simulink model "arducopter"  (R2024b)
settings: Solver=FixedStepAuto  StartTime=0.0  StopTime=simIn.param.timeEnd  FixedStep=simIn.param.dt  RelTol=1e-3
undefined symbols (not defined in the file or in its folder): DiscIntNeverNeededParam, sim, simIn
libraries: simulink x60, slident x4, vrlib x1
(part 2 of 9)

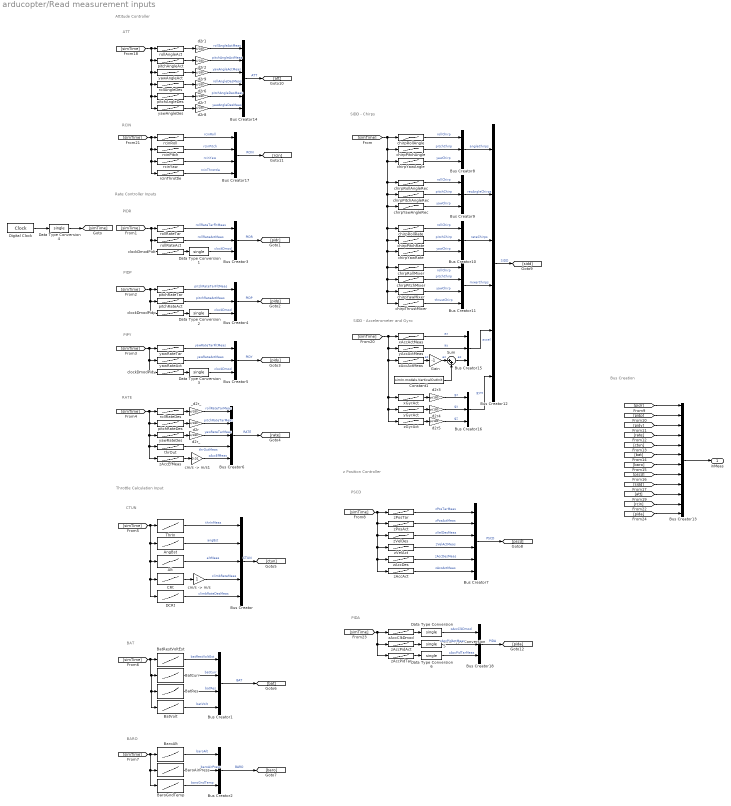
== system arducopter/Read measurement inputs ==
  note: PIDA
  note: Rate Controller Inputs
  note: SIDD - Chirps
  note: PIDR
  note: PIDP
  note: PIPY
  note: RATE
  note: CTUN
  note: BAT
  note: BARO
  note: Throttle Calculation Input
  note: PSCD
  note: z Position Controller
  note: Bus Creation
  note: ATT
  note: Attitude Controller
  note: SIDD - Accelerometer and Gyro
  note: RCIN
  Alt : Lookup_n-D  NumberOfTableDimensions=1  BreakpointsForDimension1=simIn.signals.CTUN.Time  Table=simIn.signals.CTUN.Alt  TableDataTypeStr=single  InternalRulePriority=Speed  OutDataTypeStr=Inherit: Inherit from 'Table data'  RndMeth=Simplest
  AngBst : Lookup_n-D  NumberOfTableDimensions=1  BreakpointsForDimension1=simIn.signals.CTUN.Time  Table=simIn.signals.CTUN.AngBst  TableDataTypeStr=single  InternalRulePriority=Speed  OutDataTypeStr=Inherit: Inherit from 'Table data'  RndMeth=Simplest
  BaroAirPress : Lookup_n-D  NumberOfTableDimensions=1  BreakpointsForDimension1=simIn.signals.BARO.Time  Table=simIn.signals.BARO.AirPress  TableDataTypeStr=Inherit: Inherit from 'Table data'  InternalRulePriority=Speed  OutDataTypeStr=Inherit: Inherit from 'Table data'  RndMeth=Simplest
  BaroAlt : Lookup_n-D  NumberOfTableDimensions=1  BreakpointsForDimension1=simIn.signals.BARO.Time  Table=simIn.signals.BARO.Alt  TableDataTypeStr=Inherit: Inherit from 'Table data'  InternalRulePriority=Speed  OutDataTypeStr=Inherit: Inherit from 'Table data'  RndMeth=Simplest
  BaroGndTemp : Lookup_n-D  NumberOfTableDimensions=1  BreakpointsForDimension1=simIn.signals.BARO.Time  Table=simIn.signals.BARO.GndTemp  TableDataTypeStr=Inherit: Inherit from 'Table data'  InternalRulePriority=Speed  OutDataTypeStr=Inherit: Inherit from 'Table data'  RndMeth=Simplest
  BatCurr : Lookup_n-D  NumberOfTableDimensions=1  BreakpointsForDimension1=simIn.signals.BAT.Time  Table=simIn.signals.BAT.Curr  TableDataTypeStr=single  InternalRulePriority=Speed  OutDataTypeStr=Inherit: Inherit from 'Table data'  RndMeth=Simplest
  BatRes : Lookup_n-D  NumberOfTableDimensions=1  BreakpointsForDimension1=simIn.signals.BAT.Time  Table=simIn.signals.BAT.Res  TableDataTypeStr=single  InternalRulePriority=Speed  OutDataTypeStr=Inherit: Inherit from 'Table data'  RndMeth=Simplest
  BatRestVoltEst : Lookup_n-D  NumberOfTableDimensions=1  BreakpointsForDimension1=simIn.signals.BAT.Time  Table=simIn.signals.BAT.RestVoltEst  TableDataTypeStr=single  InternalRulePriority=Speed  OutDataTypeStr=Inherit: Inherit from 'Table data'  RndMeth=Simplest
  BatVolt : Lookup_n-D  NumberOfTableDimensions=1  BreakpointsForDimension1=simIn.signals.BAT.Time  Table=simIn.signals.BAT.Volt  TableDataTypeStr=Inherit: Inherit from 'Table data'  InternalRulePriority=Speed  OutDataTypeStr=Inherit: Inherit from 'Table data'  RndMeth=Simplest
  Bus Creator : BusCreator  Inputs=5
  Bus Creator1 : BusCreator  Inputs=4
  Bus Creator{2..5,8..10,15..16,18} (10 alike) : BusCreator  Inputs=3
  Bus Creator11 : BusCreator  Inputs=4
  Bus Creator12 : BusCreator  Inputs=6
  Bus Creator13 : BusCreator  Inputs=12
  Bus Creator14 : BusCreator  Inputs=6
  Bus Creator17 : BusCreator  Inputs=4
  Bus Creator6 : BusCreator  Inputs=5
  Bus Creator7 : BusCreator  Inputs=6
  CRt : Lookup_n-D  NumberOfTableDimensions=1  BreakpointsForDimension1=simIn.signals.CTUN.Time  Table=simIn.signals.CTUN.CRt  TableDataTypeStr=single  InternalRulePriority=Speed  OutDataTypeStr=Inherit: Inherit from 'Table data'  RndMeth=Simplest
  Constant1 : Constant  Value=simIn.models.VerticalOutInit
  DCRt : Lookup_n-D  NumberOfTableDimensions=1  BreakpointsForDimension1=simIn.signals.CTUN.Time  Table=simIn.signals.CTUN.DCRt  TableDataTypeStr=single  InternalRulePriority=Speed  OutDataTypeStr=Inherit: Inherit from 'Table data'  RndMeth=Simplest
  Data Type Conversion{,1..6} (7 alike) : DataTypeConversion  OutDataTypeStr=single  SaturateOnIntegerOverflow=off  RndMeth=Floor
  Digital Clock : DigitalClock  SampleTime=simIn.param.dt
  Gain : Gain  Gain=-1
  Sum : Sum  Inputs=|++
  ThrIn : Lookup_n-D  NumberOfTableDimensions=1  BreakpointsForDimension1=simIn.signals.CTUN.Time  Table=simIn.signals.CTUN.ThrIn  TableDataTypeStr=single  InternalRulePriority=Speed  OutDataTypeStr=Inherit: Inherit from 'Table data'  RndMeth=Simplest
  _d2r_ : Gain  Gain=pi/180
  chirpPitchAngle : Lookup_n-D  NumberOfTableDimensions=1  BreakpointsForDimension1=simIn.signals.SIDD.Time{2}  Table=simIn.signals.SIDD.Chirp{2}  TableDataTypeStr=Inherit: Inherit from 'Table data'  InternalRulePriority=Speed  OutDataTypeStr=Inherit: Inherit from 'Table data'  RndMeth=Simplest
  chirpPitchAngleRec : Lookup_n-D  NumberOfTableDimensions=1  BreakpointsForDimension1=simIn.signals.SIDD.Time{5}  Table=simIn.signals.SIDD.Chirp{5}  TableDataTypeStr=Inherit: Inherit from 'Table data'  InternalRulePriority=Speed  OutDataTypeStr=Inherit: Inherit from 'Table data'  RndMeth=Simplest
  chirpPitchMixer : Lookup_n-D  NumberOfTableDimensions=1  BreakpointsForDimension1=simIn.signals.SIDD.Time{11}  Table=simIn.signals.SIDD.Chirp{11}  TableDataTypeStr=Inherit: Inherit from 'Table data'  InternalRulePriority=Speed  OutDataTypeStr=Inherit: Inherit from 'Table data'  RndMeth=Simplest
  chirpPitchRate : Lookup_n-D  NumberOfTableDimensions=1  BreakpointsForDimension1=simIn.signals.SIDD.Time{8}  Table=simIn.signals.SIDD.Chirp{8}  TableDataTypeStr=Inherit: Inherit from 'Table data'  InternalRulePriority=Speed  OutDataTypeStr=Inherit: Inherit from 'Table data'  RndMeth=Simplest
  chirpRollAngle : Lookup_n-D  NumberOfTableDimensions=1  BreakpointsForDimension1=simIn.signals.SIDD.Time{1}  Table=simIn.signals.SIDD.Chirp{1}  TableDataTypeStr=Inherit: Inherit from 'Table data'  InternalRulePriority=Speed  OutDataTypeStr=Inherit: Inherit from 'Table data'  RndMeth=Simplest
  chirpRollAngleRec : Lookup_n-D  NumberOfTableDimensions=1  BreakpointsForDimension1=simIn.signals.SIDD.Time{4}  Table=simIn.signals.SIDD.Chirp{4}  TableDataTypeStr=Inherit: Inherit from 'Table data'  InternalRulePriority=Speed  OutDataTypeStr=Inherit: Inherit from 'Table data'  RndMeth=Simplest
  chirpRollMixer : Lookup_n-D  NumberOfTableDimensions=1  BreakpointsForDimension1=simIn.signals.SIDD.Time{10}  Table=simIn.signals.SIDD.Chirp{10}  TableDataTypeStr=Inherit: Inherit from 'Table data'  InternalRulePriority=Speed  OutDataTypeStr=Inherit: Inherit from 'Table data'  RndMeth=Simplest
  chirpRollRate : Lookup_n-D  NumberOfTableDimensions=1  BreakpointsForDimension1=simIn.signals.SIDD.Time{7}  Table=simIn.signals.SIDD.Chirp{7}  TableDataTypeStr=Inherit: Inherit from 'Table data'  InternalRulePriority=Speed  OutDataTypeStr=Inherit: Inherit from 'Table data'  RndMeth=Simplest
  chirpThrustMixer : Lookup_n-D  NumberOfTableDimensions=1  BreakpointsForDimension1=simIn.signals.SIDD.Time{13}  Table=simIn.signals.SIDD.Chirp{13}  TableDataTypeStr=Inherit: Inherit from 'Table data'  InternalRulePriority=Speed  OutDataTypeStr=Inherit: Inherit from 'Table data'  RndMeth=Simplest
  chirpYawAngle : Lookup_n-D  NumberOfTableDimensions=1  BreakpointsForDimension1=simIn.signals.SIDD.Time{3}  Table=simIn.signals.SIDD.Chirp{3}  TableDataTypeStr=Inherit: Inherit from 'Table data'  InternalRulePriority=Speed  OutDataTypeStr=Inherit: Inherit from 'Table data'  RndMeth=Simplest
  chirpYawAngleRec : Lookup_n-D  NumberOfTableDimensions=1  BreakpointsForDimension1=simIn.signals.SIDD.Time{6}  Table=simIn.signals.SIDD.Chirp{6}  TableDataTypeStr=Inherit: Inherit from 'Table data'  InternalRulePriority=Speed  OutDataTypeStr=Inherit: Inherit from 'Table data'  RndMeth=Simplest
  chirpYawMixer : Lookup_n-D  NumberOfTableDimensions=1  BreakpointsForDimension1=simIn.signals.SIDD.Time{12}  Table=simIn.signals.SIDD.Chirp{12}  TableDataTypeStr=Inherit: Inherit from 'Table data'  InternalRulePriority=Speed  OutDataTypeStr=Inherit: Inherit from 'Table data'  RndMeth=Simplest
  chirpYawRate : Lookup_n-D  NumberOfTableDimensions=1  BreakpointsForDimension1=simIn.signals.SIDD.Time{9}  Table=simIn.signals.SIDD.Chirp{9}  TableDataTypeStr=Inherit: Inherit from 'Table data'  InternalRulePriority=Speed  OutDataTypeStr=Inherit: Inherit from 'Table data'  RndMeth=Simplest
  clockDmodPidp : Lookup_n-D  NumberOfTableDimensions=1  BreakpointsForDimension1=simIn.signals.PIDP.Time  Table=simIn.signals.PIDP.ClockDMod  InternalRulePriority=Speed  RndMeth=Simplest
  clockDmodPidr : Lookup_n-D  NumberOfTableDimensions=1  BreakpointsForDimension1=simIn.signals.PIDR.Time  Table=simIn.signals.PIDR.ClockDMod  TableDataTypeStr=Inherit: Inherit from 'Table data'  InternalRulePriority=Speed  OutDataTypeStr=Inherit: Inherit from 'Table data'  RndMeth=Simplest
  clockDmodPidy : Lookup_n-D  NumberOfTableDimensions=1  BreakpointsForDimension1=simIn.signals.PIDY.Time  Table=simIn.signals.PIDY.ClockDMod  InternalRulePriority=Speed  RndMeth=Simplest
  "cm/s -> m/s" : Gain
  "cm/s -> m/s1" : Gain  Gain=0.01
  d2r{,1..9} (10 alike) : Gain  Gain=pi/180
  d2r_ : Gain  Gain=pi/180
  pitchAngleAct : Lookup_n-D  NumberOfTableDimensions=1  BreakpointsForDimension1=simIn.signals.ATT.Time  Table=simIn.signals.ATT.Pitch  TableDataTypeStr=Inherit: Inherit from 'Table data'  InternalRulePriority=Speed  OutDataTypeStr=Inherit: Inherit from 'Table data'  RndMeth=Simplest
  pitchAngleDes : Lookup_n-D  NumberOfTableDimensions=1  BreakpointsForDimension1=simIn.signals.ATT.Time  Table=simIn.signals.ATT.DesPitch  TableDataTypeStr=Inherit: Inherit from 'Table data'  InternalRulePriority=Speed  OutDataTypeStr=Inherit: Inherit from 'Table data'  RndMeth=Simplest
  pitchRateAct : Lookup_n-D  NumberOfTableDimensions=1  BreakpointsForDimension1=simIn.signals.PIDP.Time  Table=simIn.signals.PIDP.Act  TableDataTypeStr=Inherit: Inherit from 'Table data'  InternalRulePriority=Speed  OutDataTypeStr=Inherit: Inherit from 'Table data'  RndMeth=Simplest
  pitchRateDes : Lookup_n-D  NumberOfTableDimensions=1  BreakpointsForDimension1=simIn.signals.RATE.Time  Table=simIn.signals.RATE.PDes  TableDataTypeStr=Inherit: Inherit from 'Table data'  InternalRulePriority=Speed  OutDataTypeStr=Inherit: Inherit from 'Table data'  RndMeth=Simplest
  pitchRateTar : Lookup_n-D  NumberOfTableDimensions=1  BreakpointsForDimension1=simIn.signals.PIDP.Time  Table=simIn.signals.PIDP.Tar  TableDataTypeStr=Inherit: Inherit from 'Table data'  InternalRulePriority=Speed  OutDataTypeStr=Inherit: Inherit from 'Table data'  RndMeth=Simplest
  rcinPitch : Lookup_n-D  NumberOfTableDimensions=1  BreakpointsForDimension1=simIn.signals.RCIN.Time  Table=simIn.signals.RCIN.PitchInput  InterpMethod=Linear Lagrange  ExtrapMethod=Clip  InternalRulePriority=Speed  OutDataTypeStr=Inherit: Inherit from 'Table data'  RndMeth=Simplest
  rcinRoll : Lookup_n-D  NumberOfTableDimensions=1  BreakpointsForDimension1=simIn.signals.RCIN.Time  Table=simIn.signals.RCIN.RollInput  TableDataTypeStr=Inherit: Inherit from 'Table data'  ExtrapMethod=Clip  InternalRulePriority=Speed  OutDataTypeStr=Inherit: Inherit from 'Table data'  RndMeth=Simplest
  rcinThrottle : Lookup_n-D  NumberOfTableDimensions=1  BreakpointsForDimension1=simIn.signals.RCIN.Time  Table=simIn.signals.RCIN.ThrottleInput  TableDataTypeStr=Inherit: Inherit from 'Table data'  ExtrapMethod=Clip  InternalRulePriority=Speed  OutDataTypeStr=Inherit: Inherit from 'Table data'  RndMeth=Simplest
  rcinYaw : Lookup_n-D  NumberOfTableDimensions=1  BreakpointsForDimension1=simIn.signals.RCIN.Time  Table=simIn.signals.RCIN.YawInput  ExtrapMethod=Clip  InternalRulePriority=Speed  OutDataTypeStr=Inherit: Inherit from 'Table data'  RndMeth=Simplest
  rollAngleAct : Lookup_n-D  NumberOfTableDimensions=1  BreakpointsForDimension1=simIn.signals.ATT.Time  Table=simIn.signals.ATT.Roll  TableDataTypeStr=Inherit: Inherit from 'Table data'  InternalRulePriority=Speed  OutDataTypeStr=Inherit: Inherit from 'Table data'  RndMeth=Simplest
  rollAngleDes : Lookup_n-D  NumberOfTableDimensions=1  BreakpointsForDimension1=simIn.signals.ATT.Time  Table=simIn.signals.ATT.DesRoll  TableDataTypeStr=Inherit: Inherit from 'Table data'  InternalRulePriority=Speed  OutDataTypeStr=Inherit: Inherit from 'Table data'  RndMeth=Simplest
  rollRateAct : Lookup_n-D  NumberOfTableDimensions=1  BreakpointsForDimension1=simIn.signals.PIDR.Time  Table=simIn.signals.PIDR.Act  TableDataTypeStr=Inherit: Inherit from 'Table data'  InternalRulePriority=Speed  OutDataTypeStr=Inherit: Inherit from 'Table data'  RndMeth=Simplest
  rollRateDes : Lookup_n-D  NumberOfTableDimensions=1  BreakpointsForDimension1=simIn.signals.RATE.Time  Table=simIn.signals.RATE.RDes  TableDataTypeStr=Inherit: Inherit from 'Table data'  InternalRulePriority=Speed  OutDataTypeStr=Inherit: Inherit from 'Table data'  RndMeth=Simplest
  rollRateTar : Lookup_n-D  NumberOfTableDimensions=1  BreakpointsForDimension1=simIn.signals.PIDR.Time  Table=simIn.signals.PIDR.Tar  TableDataTypeStr=Inherit: Inherit from 'Table data'  InternalRulePriority=Speed  OutDataTypeStr=Inherit: Inherit from 'Table data'  RndMeth=Simplest
  thrOut : Lookup_n-D  NumberOfTableDimensions=1  BreakpointsForDimension1=simIn.signals.RATE.Time  Table=simIn.signals.RATE.AOut  TableDataTypeStr=Inherit: Inherit from 'Table data'  InternalRulePriority=Speed  OutDataTypeStr=Inherit: Inherit from 'Table data'  RndMeth=Simplest
  xAccActMeas : Lookup_n-D  NumberOfTableDimensions=1  BreakpointsForDimension1=simIn.signals.SIDD.Time{1}  Table=simIn.signals.SIDD.AccX  TableDataTypeStr=Inherit: Inherit from 'Table data'  InternalRulePriority=Speed  OutDataTypeStr=Inherit: Inherit from 'Table data'  RndMeth=Simplest
  xGyrAct : Lookup_n-D  NumberOfTableDimensions=1  BreakpointsForDimension1=simIn.signals.SIDD.Time{1}  Table=simIn.signals.SIDD.GyrX  TableDataTypeStr=Inherit: Inherit from 'Table data'  InternalRulePriority=Speed  OutDataTypeStr=Inherit: Inherit from 'Table data'  RndMeth=Simplest
  yAccActMeas : Lookup_n-D  NumberOfTableDimensions=1  BreakpointsForDimension1=simIn.signals.SIDD.Time{1}  Table=simIn.signals.SIDD.AccY  TableDataTypeStr=Inherit: Inherit from 'Table data'  InternalRulePriority=Speed  OutDataTypeStr=Inherit: Inherit from 'Table data'  RndMeth=Simplest
  yGyrAct : Lookup_n-D  NumberOfTableDimensions=1  BreakpointsForDimension1=simIn.signals.SIDD.Time{1}  Table=simIn.signals.SIDD.GyrY  TableDataTypeStr=Inherit: Inherit from 'Table data'  InternalRulePriority=Speed  OutDataTypeStr=Inherit: Inherit from 'Table data'  RndMeth=Simplest
  yawAngleAct : Lookup_n-D  NumberOfTableDimensions=1  BreakpointsForDimension1=simIn.signals.ATT.Time  Table=simIn.signals.ATT.Yaw  TableDataTypeStr=Inherit: Inherit from 'Table data'  InternalRulePriority=Speed  OutDataTypeStr=Inherit: Inherit from 'Table data'  RndMeth=Simplest
  yawAngleDes : Lookup_n-D  NumberOfTableDimensions=1  BreakpointsForDimension1=simIn.signals.ATT.Time  Table=simIn.signals.ATT.DesYaw  TableDataTypeStr=Inherit: Inherit from 'Table data'  InternalRulePriority=Speed  OutDataTypeStr=Inherit: Inherit from 'Table data'  RndMeth=Simplest
  yawRateAct : Lookup_n-D  NumberOfTableDimensions=1  BreakpointsForDimension1=simIn.signals.PIDY.Time  Table=simIn.signals.PIDY.Act  TableDataTypeStr=Inherit: Inherit from 'Table data'  InternalRulePriority=Speed  OutDataTypeStr=Inherit: Inherit from 'Table data'  RndMeth=Simplest
  yawRateDes : Lookup_n-D  NumberOfTableDimensions=1  BreakpointsForDimension1=simIn.signals.RATE.Time  Table=simIn.signals.RATE.YDes  TableDataTypeStr=Inherit: Inherit from 'Table data'  InternalRulePriority=Speed  OutDataTypeStr=Inherit: Inherit from 'Table data'  RndMeth=Simplest
  yawRateTar : Lookup_n-D  NumberOfTableDimensions=1  BreakpointsForDimension1=simIn.signals.PIDY.Time  Table=simIn.signals.PIDY.Tar  TableDataTypeStr=Inherit: Inherit from 'Table data'  InternalRulePriority=Speed  OutDataTypeStr=Inherit: Inherit from 'Table data'  RndMeth=Simplest
  zAccAct : Lookup_n-D  NumberOfTableDimensions=1  BreakpointsForDimension1=simIn.signals.PSCD.Time  Table=simIn.signals.PSCD.zAccAct  TableDataTypeStr=single  InternalRulePriority=Speed  OutDataTypeStr=Inherit: Inherit from 'Table data'  RndMeth=Simplest
  zAccActMeas : Lookup_n-D  NumberOfTableDimensions=1  BreakpointsForDimension1=simIn.signals.SIDD.Time{1}  Table=simIn.signals.SIDD.AccZ  TableDataTypeStr=Inherit: Inherit from 'Table data'  InternalRulePriority=Speed  OutDataTypeStr=Inherit: Inherit from 'Table data'  RndMeth=Simplest
  zAccClkDmod : Lookup_n-D  NumberOfTableDimensions=1  BreakpointsForDimension1=simIn.signals.PIDA.Time  Table=simIn.signals.PIDA.ClockDMod  InternalRulePriority=Speed  RndMeth=Simplest
  zAccDes : Lookup_n-D  NumberOfTableDimensions=1  BreakpointsForDimension1=simIn.signals.PSCD.Time  Table=simIn.signals.PSCD.zAccDes  TableDataTypeStr=single  InternalRulePriority=Speed  OutDataTypeStr=Inherit: Inherit from 'Table data'  RndMeth=Simplest
  zAccEfMeas : Lookup_n-D  NumberOfTableDimensions=1  BreakpointsForDimension1=simIn.signals.RATE.Time  Table=simIn.signals.RATE.A  TableDataTypeStr=Inherit: Inherit from 'Table data'  InternalRulePriority=Speed  OutDataTypeStr=Inherit: Inherit from 'Table data'  RndMeth=Simplest
  zAccPidAct : Lookup_n-D  NumberOfTableDimensions=1  BreakpointsForDimension1=simIn.signals.PIDA.Time  Table=simIn.signals.PIDA.Act  InternalRulePriority=Speed  RndMeth=Simplest
  zAccPidTar : Lookup_n-D  NumberOfTableDimensions=1  BreakpointsForDimension1=simIn.signals.PIDA.Time  Table=simIn.signals.PIDA.Tar  InternalRulePriority=Speed  RndMeth=Simplest
  zGyrAct : Lookup_n-D  NumberOfTableDimensions=1  BreakpointsForDimension1=simIn.signals.SIDD.Time{1}  Table=simIn.signals.SIDD.GyrZ  TableDataTypeStr=Inherit: Inherit from 'Table data'  InternalRulePriority=Speed  OutDataTypeStr=Inherit: Inherit from 'Table data'  RndMeth=Simplest
  zPosAct : Lookup_n-D  NumberOfTableDimensions=1  BreakpointsForDimension1=simIn.signals.PSCD.Time  Table=simIn.signals.PSCD.zPosAct  TableDataTypeStr=single  InternalRulePriority=Speed  OutDataTypeStr=Inherit: Inherit from 'Table data'  RndMeth=Simplest
  zPosTar : Lookup_n-D  NumberOfTableDimensions=1  BreakpointsForDimension1=simIn.signals.PSCD.Time  Table=simIn.signals.PSCD.zPosTar  TableDataTypeStr=single  InternalRulePriority=Speed  OutDataTypeStr=Inherit: Inherit from 'Table data'  RndMeth=Simplest
  zVelAct : Lookup_n-D  NumberOfTableDimensions=1  BreakpointsForDimension1=simIn.signals.PSCD.Time  Table=simIn.signals.PSCD.zVelAct  TableDataTypeStr=Inherit: Inherit from 'Table data'  InternalRulePriority=Speed  OutDataTypeStr=single  RndMeth=Simplest
  zVelDes : Lookup_n-D  NumberOfTableDimensions=1  BreakpointsForDimension1=simIn.signals.PSCD.Time  Table=simIn.signals.PSCD.zVelDes  TableDataTypeStr=single  InternalRulePriority=Speed  OutDataTypeStr=Inherit: Inherit from 'Table data'  RndMeth=Simplest
  inMeas : Outport
  wires:
  Digital Clock/1 -> Data Type Conversion4/1
  [simTime] -> chirpThrustMixer/1, chirpYawMixer/1, chirpPitchMixer/1, chirpRollMixer/1, chirpYawRate/1, chirpPitchRate/1, chirpRollRate/1, chirpYawAngleRec/1, chirpPitchAngleRec/1, chirpRollAngleRec/1, chirpYawAngle/1, chirpPitchAngle/1, chirpRollAngle/1
  [simTime] -> clockDmodPidr/1, rollRateAct/1, rollRateTar/1
  [simTime] -> clockDmodPidp/1, pitchRateAct/1, pitchRateTar/1
  [simTime] -> yawRateAct/1, clockDmodPidy/1, yawRateTar/1
  [simTime] -> rollRateDes/1, zAccEfMeas/1, thrOut/1, yawRateDes/1, pitchRateDes/1
  ThrIn/1 -> Bus Creator/1  "thrInMeas"
  BaroAlt/1 -> Bus Creator2/1  "baroAlt"
  BaroAirPress/1 -> Bus Creator2/2  "baroAirPress"
  AngBst/1 -> Bus Creator/2  "angBst"
  BatCurr/1 -> Bus Creator1/2  "batCurr"
  BatVolt/1 -> Bus Creator1/4  "batVolt"
  BaroGndTemp/1 -> Bus Creator2/3  "baroGndTemp"
  BatRes/1 -> Bus Creator1/3  "batRes"
  BatRestVoltEst/1 -> Bus Creator1/1  "batRestVoltEst"
  [simTime] -> CRt/1, DCRt/1, Alt/1, AngBst/1, ThrIn/1
  [simTime] -> BatVolt/1, BatRes/1, BatCurr/1, BatRestVoltEst/1
  [simTime] -> BaroGndTemp/1, BaroAirPress/1, BaroAlt/1
  rollRateTar/1 -> Bus Creator3/1  "rollRateTarFltMeas"
  clockDmodPidr/1 -> Data Type Conversion1/1
  pitchRateTar/1 -> Bus Creator4/1  "pitchRateTarFltMeas"
  clockDmodPidp/1 -> Data Type Conversion2/1
  yawRateAct/1 -> Bus Creator5/2  "yawRateActMeas"
  yawRateTar/1 -> Bus Creator5/1  "yawRateTarFltMeas"
  clockDmodPidy/1 -> Data Type Conversion3/1
  pitchRateDes/1 -> d2r/1
  rollRateDes/1 -> _d2r_/1
  yawRateDes/1 -> d2r_/1
  d2r_/1 -> Bus Creator6/3  "yawRateTarMeas"
  Bus Creator3/1 -> [pidr]  "PIDR"
  Bus Creator4/1 -> [pidp]  "PIDP"
  Bus Creator5/1 -> [pidy]  "PIDY"
  Bus Creator6/1 -> [rate]  "RATE"
  Bus Creator/1 -> [ctun]  "CTUN"
  Bus Creator1/1 -> [bat]  "BAT"
  Bus Creator2/1 -> [baro]  "BARO"
  zPosAct/1 -> Bus Creator7/2  "zPosActMeas"
  zVelDes/1 -> Bus Creator7/3  "zVelDesMeas"
  zVelAct/1 -> Bus Creator7/4  "zVelActMeas"
  zAccAct/1 -> Bus Creator7/6  "zAccActMeas"
  zPosTar/1 -> Bus Creator7/1  "zPosTarMeas"
  zAccDes/1 -> Bus Creator7/5  "zAccDesMeas"
  [simTime] -> zPosAct/1, zAccAct/1, zAccDes/1, zVelAct/1, zVelDes/1, zPosTar/1
  Bus Creator7/1 -> [pscd]  "PSCD"
  Data Type Conversion1/1 -> Bus Creator3/3  "clockDmod"
  Data Type Conversion2/1 -> Bus Creator4/3  "clockDmod"
  Data Type Conversion3/1 -> Bus Creator5/3  "clockDmod"
  chirpPitchAngle/1 -> Bus Creator8/2  "pitchChirp"
  chirpRollAngle/1 -> Bus Creator8/1  "rollChirp"
  chirpYawAngle/1 -> Bus Creator8/3  "yawChirp"
  Bus Creator8/1 -> Bus Creator12/1  "angleChirps"
  chirpPitchAngleRec/1 -> Bus Creator9/2  "pitchChirp"
  chirpRollAngleRec/1 -> Bus Creator9/1  "rollChirp"
  chirpYawAngleRec/1 -> Bus Creator9/3  "yawChirp"
  Bus Creator9/1 -> Bus Creator12/2  "recAngleChirps"
  chirpPitchRate/1 -> Bus Creator10/2  "pitchChirp"
  chirpRollRate/1 -> Bus Creator10/1  "rollChirp"
  chirpYawRate/1 -> Bus Creator10/3  "yawChirp"
  Bus Creator10/1 -> Bus Creator12/3  "rateChirps"
  chirpRollMixer/1 -> Bus Creator11/1  "rollChirp"
  chirpPitchMixer/1 -> Bus Creator11/2  "pitchChirp"
  chirpYawMixer/1 -> Bus Creator11/3  "yawChirp"
  Bus Creator11/1 -> Bus Creator12/4  "mixerChirps"
  chirpThrustMixer/1 -> Bus Creator11/4  "thrustChirp"
  Bus Creator12/1 -> [sidd]  "SIDD"
  Bus Creator13/1 -> inMeas/1
  [pidr] -> Bus Creator13/1
  [pidp] -> Bus Creator13/2
  [pidy] -> Bus Creator13/3
  [rate] -> Bus Creator13/4
  [ctun] -> Bus Creator13/5
  [bat] -> Bus Creator13/6
  [baro] -> Bus Creator13/7
  [pscd] -> Bus Creator13/8
  [sidd] -> Bus Creator13/9
  Data Type Conversion4/1 -> [simTime]
  pitchRateAct/1 -> Bus Creator4/2  "pitchRateActMeas"
  _d2r_/1 -> Bus Creator6/1  "rollRateTarMeas"
  rollRateAct/1 -> Bus Creator3/2  "rollRateActMeas"
  d2r/1 -> Bus Creator6/2  "pitchRateTarMeas"
  d2r2/1 -> Bus Creator14/2  "pitchAngleActMeas"
  Bus Creator14/1 -> [att]  "ATT"
  d2r1/1 -> Bus Creator14/1  "rollAngleActMeas"
  [simTime] -> rollAngleAct/1, yawAngleAct/1, yawAngleDes/1, pitchAngleDes/1, rollAngleDes/1, pitchAngleAct/1
  [att] -> Bus Creator13/10
  [simTime] -> zGyrAct/1, yGyrAct/1, xGyrAct/1, zAccActMeas/1, yAccActMeas/1, xAccActMeas/1
  xAccActMeas/1 -> Bus Creator15/1  "ax"
  yAccActMeas/1 -> Bus Creator15/2  "ay"
  xGyrAct/1 -> d2r3/1
  yGyrAct/1 -> d2r4/1
  zGyrAct/1 -> d2r5/1
  Bus Creator15/1 -> Bus Creator12/5  "accel"
  Bus Creator16/1 -> Bus Creator12/6  "gyro"
  rollAngleAct/1 -> d2r1/1
  pitchAngleAct/1 -> d2r2/1
  d2r3/1 -> Bus Creator16/1  "gx"
  d2r4/1 -> Bus Creator16/2  "gy"
  d2r5/1 -> Bus Creator16/3  "gz"
  pitchAngleDes/1 -> d2r7/1
  rollAngleDes/1 -> d2r6/1
  d2r6/1 -> Bus Creator14/4  "rollAngleDesMeas"
  d2r7/1 -> Bus Creator14/5  "pitchAngleDesMeas"
  yawAngleDes/1 -> d2r8/1
  d2r8/1 -> Bus Creator14/6  "yawAngleDesMeas"
  yawAngleAct/1 -> d2r9/1
  d2r9/1 -> Bus Creator14/3  "yawAngleActMeas"
  rcinRoll/1 -> Bus Creator17/1  "rcinRoll"
  rcinPitch/1 -> Bus Creator17/2  "rcinPitch"
  rcinYaw/1 -> Bus Creator17/3  "rcinYaw"
  Bus Creator17/1 -> [rcin]  "RCIN"
  [rcin] -> Bus Creator13/11
  [simTime] -> rcinRoll/1, rcinThrottle/1, rcinYaw/1, rcinPitch/1
  thrOut/1 -> Bus Creator6/4  "thrOutMeas"
  zAccEfMeas/1 -> "cm/s -> m/s1"/1
  zAccActMeas/1 -> Gain/1  "az"
  Alt/1 -> Bus Creator/3  "altMeas"
  CRt/1 -> "cm/s -> m/s"/1
  "cm/s -> m/s"/1 -> Bus Creator/4  "climbRateMeas"
  Sum/1 -> Bus Creator15/3  "az"
  "cm/s -> m/s1"/1 -> Bus Creator6/5  "zAccEfMeas"
  Gain/1 -> Sum/1  "az"
  Constant1/1 -> Sum/2
  Data Type Conversion/1 -> Bus Creator18/1  "zAccClkDmod"
  zAccClkDmod/1 -> Data Type Conversion/1
  [simTime] -> zAccPidTar/1, zAccPidAct/1, zAccClkDmod/1
  zAccPidAct/1 -> Data Type Conversion5/1
  zAccPidTar/1 -> Data Type Conversion6/1
  Data Type Conversion5/1 -> Bus Creator18/2  "zAccPidActMeas"
  Data Type Conversion6/1 -> Bus Creator18/3  "zAccPidTarMeas"
  Bus Creator18/1 -> [pida]  "PIDA"
  [pida] -> Bus Creator13/12
  DCRt/1 -> Bus Creator/5  "climbRateDesMeas"
  rcinThrottle/1 -> Bus Creator17/4  "rcinThrottle"

== system arducopter/Throttle ==
  note: Throttle Calculation Outputs
  note: Throttle Calculation Inputs
  note: Simulation
  note: Measurements
  note: Sponsored by IAV GmbH
  inMeas : Inport
  thrMixOut : Inport  Port=2
  thrIn : Inport  Port=3
  zVelCtrlRatio : Inport  Port=4
  zVelDes : Inport  Port=5
  zVelAct : Inport  Port=6
  AirDensityRatioMeas : Lookup_n-D  NumberOfTableDimensions=1  BreakpointsForDimension1=simIn.signals.MOTQ.Time  Table=simIn.signals.MOTQ.CompGain  InternalRulePriority=Speed  RndMeth=Simplest
  Bus Creator4 : BusCreator  Inputs=1
  Bus Creator5 : BusCreator  Inputs=1
  Bus Selector : BusSelector  OutputSignals=thrTar,angBst,batRestVoltEst,batCurr,batRes,batVolt,baroAlt,baroAirPress,baroGndTemp
  Clock1 : Clock
  Input Handler : Subsystem
      settings: PortSchema="{\"entries\":[{\"content\":{\"sides\":[{\"content\":{\"connectorIds\":[\"In1\",\"In2\"]},\"type\":\"ConnectorPlacement.EquallySpacedRectSide\",\"uuid\":\"11925210-52ad-46bf-880a-53173efcdcd2\"},{\"content\":{\"connectorIds\":[\"Out1\"],\"side\":\"RIGHT\"},\"type\":\"ConnectorPlacement.EquallySpacedRectSide\",\"uuid\":\"6251752b-5f08-4f08-ba6e-4e858d08d357\"},{\"content\":{\"connectorIds\":[\"In3\"],\"side\":\"TOP\"},\"type\":\"ConnectorPlacement.EquallySpacedRectSide\",\"uuid\":\"3d8207f5-9b82-4b6f-a3de-4afdf5552ee4\"}]},\"type\":\"ConnectorPlacement.EquallySpacedConnector\",\"uuid\":\"c30d1dfe-4621-494f-aa68-a45db90b73bf\"}],\"packageUris\":[\"http://schema.mathworks.com/mf0/Connector/R2020b\"],\"version\":\"1.0\"}"
  LiftMaxMeas : Lookup_n-D  NumberOfTableDimensions=1  BreakpointsForDimension1=simIn.signals.MOTB.Time  Table=simIn.signals.MOTB.LiftMax  InternalRulePriority=Speed  RndMeth=Simplest
  Terminator{,1..6,9} (8 alike) : Terminator
  ThrAvgMaxMeas : Lookup_n-D  NumberOfTableDimensions=1  BreakpointsForDimension1=simIn.signals.MOTB.Time  Table=simIn.signals.MOTB.ThrAvMx  InternalRulePriority=Speed  RndMeth=Simplest
  ThrHovMeas : Lookup_n-D  NumberOfTableDimensions=1  BreakpointsForDimension1=simIn.signals.CTUN.Time  Table=simIn.signals.CTUN.ThrHov  InternalRulePriority=Speed  RndMeth=Simplest
  ThrLimitMeas : Lookup_n-D  NumberOfTableDimensions=1  BreakpointsForDimension1=simIn.signals.MOTB.Time  Table=simIn.signals.MOTB.ThrLimit  InternalRulePriority=Speed  RndMeth=Simplest
  ThrOutMeas : Lookup_n-D  NumberOfTableDimensions=1  BreakpointsForDimension1=simIn.signals.CTUN.Time  Table=simIn.signals.CTUN.ThrOut  InternalRulePriority=Speed  RndMeth=Simplest
  ThrThstMaxMeas : Lookup_n-D  NumberOfTableDimensions=1  BreakpointsForDimension1=simIn.signals.MOTQ.Time  Table=simIn.signals.MOTQ.ThrThstMaxMeas  InternalRulePriority=Speed  RndMeth=Simplest
  Throttle Calculations : Subsystem
      settings: PortSchema="{\"entries\":[{\"content\":{\"sides\":[{\"content\":{\"connectorIds\":[\"In1\",\"In2\",\"In3\",\"In4\",\"In5\",\"In6\",\"In7\",\"In8\",\"In9\",\"In10\",\"In11\",\"In12\",\"In13\"]},\"type\":\"ConnectorPlacement.EquallySpacedRectSide\",\"uuid\":\"f202da64-deee-49ff-ada4-059a359ae5f9\"},{\"content\":{\"connectorIds\":[\"Out1\",\"Out2\",\"Out3\",\"Out4\",\"Out5\",\"Out6\",\"Out7\"],\"side\":\"RIGHT\"},\"type\":\"ConnectorPlacement.EquallySpacedRectSide\",\"uuid\":\"b4cbbae5-26a8-4507-9891-ba8141ecb816\"},{\"content\":{\"connectorIds\":[\"In14\"],\"side\":\"TOP\"},\"type\":\"ConnectorPlacement.EquallySpacedRectSide\",\"uuid\":\"6cf4cc08-1bdf-442e-997b-fcd659fc037b\"}]},\"type\":\"ConnectorPlacement.EquallySpacedConnector\",\"uuid\":\"9cae1d38-7a6f-488f-b2c3-9ced97d183b2\"}],\"packageUris\":[\"http://schema.mathworks.com/mf0/Connector/R2020b\"],\"version\":\"1.0\"}"
  Throttle Manual Flag : Constant  Value=simIn.param.MODE.THR_MAN_FLG
  compGainMeas : Lookup_n-D  NumberOfTableDimensions=1  BreakpointsForDimension1=simIn.signals.MOTQ.Time  Table=simIn.signals.MOTQ.CompGain  InternalRulePriority=Speed  RndMeth=Simplest
  thrOutFilt : Outport
  thrAvgMax : Outport  Port=2
  thrThstMax : Outport  Port=3
  compGain : Outport  Port=4
  thrHover : Outport  Port=5
  altholdLeanAngleMax : Outport  Port=6
  thrSlewRate : Outport  Port=7
  wires:
  Bus Selector/4 -> Throttle Calculations/4(batCurr)  "<batCurr>"
  Throttle Calculations/2(thrAvgMax) -> thrAvgMax/1  "thrAvgMax"
  Bus Selector/8 -> Throttle Calculations/8(baroAirPress)  "<baroAirPress>"
  Bus Selector/6 -> Throttle Calculations/6(batVolt)  "<batVolt>"
  Throttle Calculations/1(thrOutFilt) -> thrOutFilt/1  "thrOutFilt"
  Bus Selector/2 -> Throttle Calculations/2(angBst)  "<angBst>"
  Bus Selector/1 -> Throttle Calculations/1(thrIn)  "<thrTar>"
  Bus Selector/7 -> Throttle Calculations/7(baroAlt)  "<baroAlt>"
  Bus Selector/3 -> Throttle Calculations/3(batRestVoltEst)  "<batRestVoltEst>"
  Bus Selector/5 -> Throttle Calculations/5(batRes)  "<batRes>"
  Throttle Calculations/3(thrThstMax) -> thrThstMax/1
  Throttle Calculations/4(comp_gain) -> compGain/1
  Throttle Calculations/5(thrHover) -> thrHover/1  "thrHover"
  thrIn/1 -> Bus Creator4/1  "thrIn"
  Bus Creator4/1 -> Bus Creator5/1  "throttle"
  Bus Creator5/1 -> [inSim]  "sim"
  [inSim] -> Input Handler/2(inSim)
  [inMeas] -> Input Handler/1(inMeas)
  Throttle Manual Flag/1 -> Throttle Calculations/14(thrMan), Input Handler/3(thrMan)
  Input Handler/1(data_in) -> Bus Selector/1
  Bus Selector/9 -> Throttle Calculations/9(baroGndTemp)  "<baroGndTemp>"
  ThrHovMeas/1 -> Terminator/1  "thrHovMeas"
  LiftMaxMeas/1 -> Terminator9/1  "liftMaxMeas"
  ThrOutMeas/1 -> Terminator6/1  "thrOutMeas"
  ThrLimitMeas/1 -> Terminator4/1  "thrLimitMeas"
  zVelCtrlRatio/1 -> [zVelCtrlRatio]
  [zVelCtrlRatio] -> Throttle Calculations/10(zVelCtrlRatio)
  zVelDes/1 -> [zVelDes]
  [zVelDes] -> Throttle Calculations/11(zVelDes)
  [zVelAct] -> Throttle Calculations/12(zVelAct)
  zVelAct/1 -> [zVelAct]
  ThrAvgMaxMeas/1 -> Terminator1/1  "thrAvgMaxMeas"
  ThrThstMaxMeas/1 -> Terminator2/1  "thrThstMaxMeas"
  compGainMeas/1 -> Terminator3/1  "compGainMeas"
  AirDensityRatioMeas/1 -> Terminator5/1  "airDensityRatioMeas"
  Clock1/1 -> ThrLimitMeas/1, ThrHovMeas/1, AirDensityRatioMeas/1, compGainMeas/1, ThrThstMaxMeas/1, ThrAvgMaxMeas/1, ThrOutMeas/1, LiftMaxMeas/1
  inMeas/1 -> [inMeas]
  thrMixOut/1 -> [thrMixOut]
  [thrMixOut] -> Throttle Calculations/13(thrMixOut)
  Throttle Calculations/6(altholdLeanAngleMax) -> altholdLeanAngleMax/1  "altholdLeanAngleMax"
  Throttle Calculations/7(thrSlewRate) -> thrSlewRate/1

== system arducopter/radioIn to controlIn ==
  note: Wo im Code finde ich, dass im Stabilize Mode Roll,Pitch als to_angle und Yaw als to_range angegeben ist.
      | Unter radio.cpp sind alle drei to_angle
      | chatgpt sagt alle werden als to_range aufgenommen und später in Winkel umgerechnet
  note: high_in = 1000, defined in Copter::init_rc_in()
  note: Calculation of control values from radio input.
      | The functions are called from pwm_to_range() or pwm_to_ange() (roll,pitch,yaw) in RC_Channel::update().
      | For the throttle channel, the pwm_to_range() function is called, since it is a range type radio channel (Copter::default_dead_zones() -> channel_throttle->set_range())
  note: norm_input_dz() in mode_stabilize.cpp control.cpp
      | Called in ModeStabilize::run() to norm the yaw radio input of the pilot
  note: Sponsored by IAV GmbH
  rcInRoll : Inport
  rcInPitch : Inport  Port=2
  rcInYaw : Inport  Port=3
  rcInThrottle : Inport  Port=4
  Constant : Constant  Value=simIn.param.RCIN.DZ_RLL
  Constant1 : Constant  Value=simIn.param.RCIN.MIN_RLL
  Constant10 : Constant  Value=simIn.param.RCIN.DZ_YAW
  Constant11 : Constant  Value=simIn.param.RCIN.MIN_YAW
  Constant12 : Constant  Value=simIn.param.RCIN.MAX_YAW
  Constant13 : Constant  Value=simIn.param.RCIN.REVERSED_YAW
  Constant15 : Constant  Value=simIn.param.RCIN.TRIM_PIT
  Constant16 : Constant  Value=simIn.param.RCIN.TRIM_YAW
  Constant17 : Constant  Value=simIn.param.RCIN.TRIM_RLL
  Constant18 : Constant  Value=simIn.param.RCIN.DZ_THR
  Constant19 : Constant  Value=simIn.param.RCIN.MIN_THR
  Constant2 : Constant  Value=simIn.param.RCIN.MAX_RLL
  Constant20 : Constant  Value=simIn.param.RCIN.MAX_THR
  Constant21 : Constant  Value=simIn.param.RCIN.REVERSED_THR
  Constant22 : Constant  Value=1000
  Constant3 : Constant  Value=simIn.param.RCIN.REVERSED_RLL
  Constant4 : Constant  Value=simIn.param.RCIN.ROLL_PITCH_YAW_INPUT_MAX
  Constant5 : Constant  Value=simIn.param.RCIN.DZ_PIT
  Constant6 : Constant  Value=simIn.param.RCIN.MIN_PIT
  Constant7 : Constant  Value=simIn.param.RCIN.MAX_PIT
  Constant8 : Constant  Value=simIn.param.RCIN.REVERSED_PIT
  Constant9 : Constant  Value=simIn.param.RCIN.ROLL_PITCH_YAW_INPUT_MAX
  MATLAB Function : MATLAB Function  TreatAsAtomicUnit=on
  MATLAB Function1 : MATLAB Function  TreatAsAtomicUnit=on
  MATLAB Function2 : MATLAB Function  TreatAsAtomicUnit=on
  MATLAB Function3 : MATLAB Function  TreatAsAtomicUnit=on
  ctrlInRoll : Outport
  ctrlInPitch : Outport  Port=2
  ctrlInYaw : Outport  Port=3
  ctrlInThrottle : Outport  Port=4
  wires:
  rcInRoll/1 -> MATLAB Function/1(rcIn)
  Constant/1 -> MATLAB Function/2(deadZone)
  Constant1/1 -> MATLAB Function/3(radioMin)
  Constant2/1 -> MATLAB Function/4(radioMax)
  Constant3/1 -> MATLAB Function/6(reversed)
  Constant4/1 -> MATLAB Function/7(highIn)
  Constant8/1 -> MATLAB Function3/6(reversed)
  Constant9/1 -> MATLAB Function3/7(highIn)
  Constant5/1 -> MATLAB Function3/2(deadZone)
  Constant6/1 -> MATLAB Function3/3(radioMin)
  Constant7/1 -> MATLAB Function3/4(radioMax)
  rcInPitch/1 -> MATLAB Function3/1(rcIn)
  rcInYaw/1 -> MATLAB Function1/1(radioIn)
  MATLAB Function/1(angleIn) -> ctrlInRoll/1
  MATLAB Function3/1(angleIn) -> ctrlInPitch/1
  MATLAB Function1/1(out) -> ctrlInYaw/1
  Constant17/1 -> MATLAB Function/5(trim)
  Constant15/1 -> MATLAB Function3/5(trim)
  MATLAB Function2/1(ctrlIn) -> ctrlInThrottle/1
  rcInThrottle/1 -> MATLAB Function2/1(rcIn)
  Constant21/1 -> MATLAB Function2/5(reversed)
  Constant19/1 -> MATLAB Function2/3(radioMin)
  Constant20/1 -> MATLAB Function2/4(radioMax)
  Constant22/1 -> MATLAB Function2/6(highIn)
  Constant18/1 -> MATLAB Function2/2(deadZone)
  Constant12/1 -> MATLAB Function1/5(radioMax)
  Constant13/1 -> MATLAB Function1/6(reversed)
  Constant10/1 -> MATLAB Function1/2(deadZone)
  Constant16/1 -> MATLAB Function1/3(radioTrim)
  Constant11/1 -> MATLAB Function1/4(radioMin)

== system arducopter/Attitude Controller/Determine angleLimit ==
  note: If mode == Althold, use calculated maximum lean angle, that is calculated in AC_AttitudeControl_Multi.cpp.
      | In all other modes, use ANGLE_MAX as done in mode_stabilize.cpp, run()
  altholdLeanAngleMax : Inport
  Compare To Constant : simulink/Logic and Bit Operations/Compare To Constant  relop===  const=2  OutDataTypeStr=boolean
  Constant4 : Constant  Value=simIn.param.ATC.ANGLE_LIMIT_MIN
  Constant5 : Constant  Value=simIn.param.ANGLE_MAX
  Constant6 : Constant  Value=simIn.param.MODE.ModeNr
  MATLAB Function2 : MATLAB Function  TreatAsAtomicUnit=on
  Switch : Switch  Criteria=u2 > Threshold  SaturateOnIntegerOverflow=off  InputSameDT=off
  angleLimit : Outport
  wires:
  altholdLeanAngleMax/1 -> MATLAB Function2/1(altholdLeanAngleMax)
  Switch/1 -> angleLimit/1
  Constant4/1 -> MATLAB Function2/2(angleLimitMin)
  Constant5/1 -> Switch/3
  Constant6/1 -> Compare To Constant/1
  MATLAB Function2/1(altholdLeanAngleMaxCDeg) -> Switch/1
  Compare To Constant/1 -> Switch/2
